simulink model "inverted_pendulum_controlled"  (R2025a)
settings: Solver=ode45  StartTime=0.0  StopTime=30  MaxStep=0.01  RelTol=1e-3
model workspace (MAT data in the model file):
  disturbance_signal = [0  0; 30.1  0]
settings Model: Creator=user  LastModifiedBy=user
settings DataIOCC: SaveOutput=off  SaveTime=off

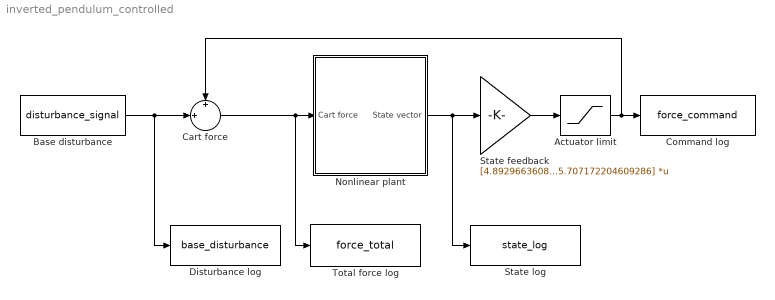
== system inverted_pendulum_controlled ==
  Actuator limit : Saturate  UpperLimit=10  LowerLimit=-10
  Base disturbance : FromWorkspace  VariableName=disturbance_signal  Interpolate=off  OutputAfterFinalValue=Holding final value
  Cart force : Sum  Inputs=+|+||
  Command log : ToWorkspace  VariableName=force_command  SaveFormat=Timeseries  SampleTime=-1
  Disturbance log : ToWorkspace  VariableName=base_disturbance  SaveFormat=Timeseries  SampleTime=-1
  Nonlinear plant : Subsystem
  State feedback : Gain  Gain=[4.8929663608562688 7.7571722046092892 85.573109804948473 25.707172204609286]  Multiplication=Matrix(K*u)
  State log : ToWorkspace  VariableName=state_log  SaveFormat=Timeseries  SampleTime=-1
  Total force log : ToWorkspace  VariableName=force_total  SaveFormat=Timeseries  SampleTime=-1
  wires:
  Base disturbance/1 -> Cart force/2, Disturbance log/1
  Cart force/1 -> Total force log/1, Nonlinear plant/1(Cart force)
  Nonlinear plant/1(State vector) -> State log/1, State feedback/1
  State feedback/1 -> Actuator limit/1
  Actuator limit/1 -> Cart force/1, Command log/1

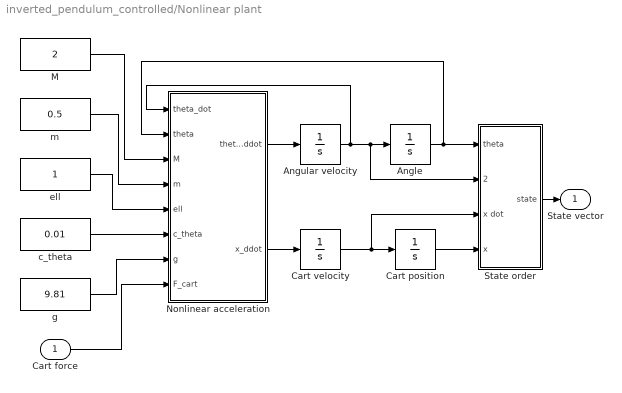
== system inverted_pendulum_controlled/Nonlinear plant ==
  Cart force : Inport
  Angle : Integrator  InitialCondition=5*pi/180
  Angular velocity : Integrator
  Cart position : Integrator
  Cart velocity : Integrator
  M : Constant  Value=2
  Nonlinear acceleration : MATLAB Function  TreatAsAtomicUnit=on
  State order : Subsystem
      mask Display: port_label('input',1,'theta');port_label('input',2,'theta dot');port_label('input',3,'x dot');port_label('input',4,'x');port_label('output',1,'state');
  c_theta : Constant  Value=0.01
  ell : Constant
  g : Constant  Value=9.81
  m : Constant  Value=0.5
  State vector : Outport
  wires:
  M/1 -> Nonlinear acceleration/3(M)
  m/1 -> Nonlinear acceleration/4(m)
  ell/1 -> Nonlinear acceleration/5(ell)
  c_theta/1 -> Nonlinear acceleration/6(c_theta)
  g/1 -> Nonlinear acceleration/7(g)
  Cart force/1 -> Nonlinear acceleration/8(F_cart)
  Nonlinear acceleration/1(theta_ddot) -> Angular velocity/1
  Nonlinear acceleration/2(x_ddot) -> Cart velocity/1
  Angular velocity/1 -> Angle/1, State order/2(theta dot), Nonlinear acceleration/1(theta_dot)
  Cart velocity/1 -> Cart position/1, State order/3(x dot)
  Angle/1 -> Nonlinear acceleration/2(theta), State order/1(theta)
  Cart position/1 -> State order/4(x)
  State order/1(state) -> State vector/1

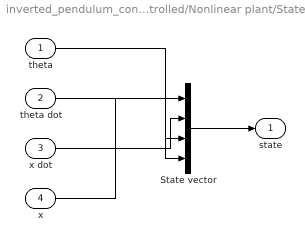
== system inverted_pendulum_controlled/Nonlinear plant/State order ==
  theta : Inport
  theta dot : Inport  Port=2
  x dot : Inport  Port=3
  x : Inport  Port=4
  State vector : Mux
  state : Outport
  wires:
  x/1 -> State vector/1
  x dot/1 -> State vector/2
  theta/1 -> State vector/3
  theta dot/1 -> State vector/4
  State vector/1 -> state/1

== matlab function inverted_pendulum_controlled/Nonlinear plant/Nonlinear acceleration ==
  data: theta_dot input; theta_ddot output; theta input; x_ddot output; M input; m input; ell input; c_theta input; g input; F_cart input
function [theta_ddot, x_ddot] = accelerations(theta_dot, theta, M, m, ell, c_theta, g, F_cart)
% Nonlinear cart-pendulum equations with an applied horizontal cart force.
% Positive theta is the upright perturbation used in Mini Project 1.

s = sin(theta);
c = cos(theta);
mass_matrix = [M + m, m * ell * c; m * ell * c, m * ell^2];
forcing = [F_cart + m * ell * s * theta_dot^2; ...
           m * g * ell * s - c_theta * theta_dot];
acceleration = mass_matrix \ forcing;

x_ddot = acceleration(1);
theta_ddot = acceleration(2);
end
